simulink model "b7476dof"  (R2024b)
settings: Solver=VariableStepAuto  StartTime=0.0  StopTime=10.0  RelTol=1e-3
settings Model: Creator=adasu  LastModifiedBy=adasu

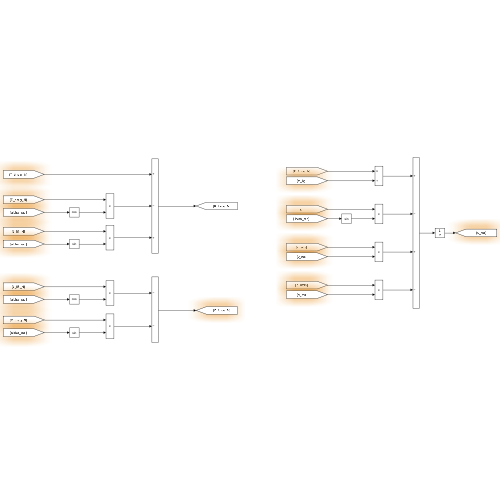
[thumbnail: Simulink's stored preview of the top-level diagram]
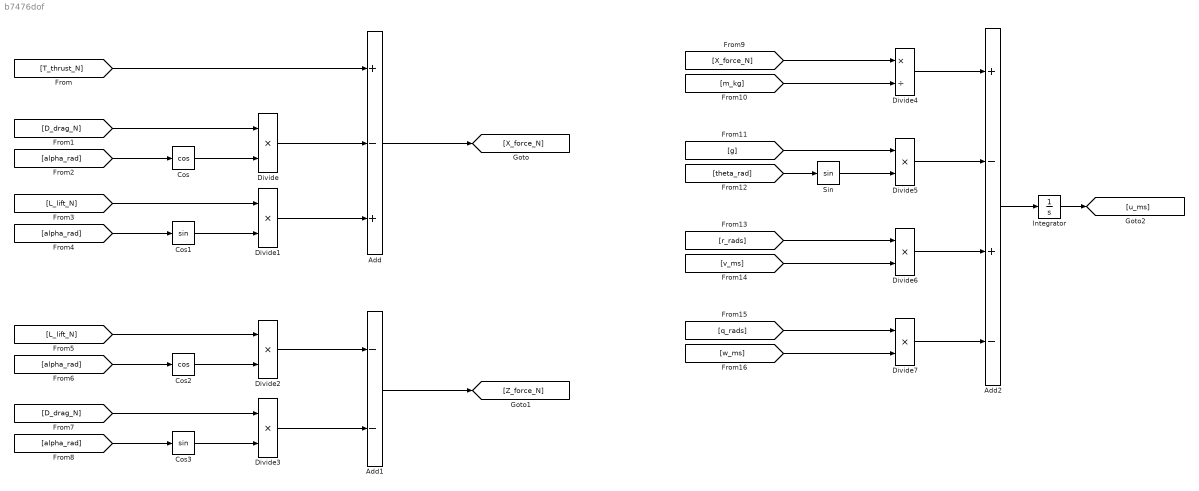
== system b7476dof ==
  Add : Sum  Inputs=+-+
  Add1 : Sum  Inputs=--
  Add2 : Sum  Inputs=+-+-
  Cos : Trigonometry  Operator=cos
  Cos1 : Trigonometry
  Cos2 : Trigonometry  Operator=cos
  Cos3 : Trigonometry
  Divide{,1..3,5..7} (7 alike) : Product  Inputs=**
  Divide4 : Product  Inputs=*/
  Integrator : Integrator
  Sin : Trigonometry
  wires:
  [D_drag_N] -> Divide/1
  [alpha_rad] -> Cos/1
  [L_lift_N] -> Divide1/1
  [alpha_rad] -> Cos1/1
  Divide1/1 -> Add/3
  Divide/1 -> Add/2
  [T_thrust_N] -> Add/1
  Add/1 -> [X_force_N]
  Cos/1 -> Divide/2
  Cos1/1 -> Divide1/2
  [alpha_rad] -> Cos2/1
  [L_lift_N] -> Divide2/1
  Cos2/1 -> Divide2/2
  [alpha_rad] -> Cos3/1
  Cos3/1 -> Divide3/2
  [D_drag_N] -> Divide3/1
  Divide2/1 -> Add1/1
  Divide3/1 -> Add1/2
  Add1/1 -> [Z_force_N]
  [X_force_N] -> Divide4/1
  [m_kg] -> Divide4/2
  [theta_rad] -> Sin/1
  Sin/1 -> Divide5/2
  [g] -> Divide5/1
  [r_rads] -> Divide6/1
  [v_ms] -> Divide6/2
  [w_ms] -> Divide7/2
  [q_rads] -> Divide7/1
  Divide7/1 -> Add2/4
  Divide6/1 -> Add2/3
  Divide5/1 -> Add2/2
  Divide4/1 -> Add2/1
  Add2/1 -> Integrator/1
  Integrator/1 -> [u_ms]
